simulink model "afe_dqctrl_inv_psm"  (R2026a)
settings: Solver=ode23t  StopTime=simlength  FixedStep=tc  MaxStep=glb_time.tc  RelTol=1e-4
values from neighbouring files (symbols this model uses):
  afe_ctrl = ctrl_afe_setup(glb_time.ts_afe, grid_emu.omega_grid_nom)    [init_model.m]
  afe_pwm_phase_shift_mod1 = 0    [init_model.m]
  CTRPIFF_CLIP_RELEASE = 0.001    [init_model.m]
  filters = setup_global_filters(glb_time.ts_afe, glb_time.ts_inv, glb_time.ts_dab, glb_time.tc)    [init_model.m]
  glb_time = timing_setup(fpwm_afe, trgo_afe, fpwm_inv, trgo_inv, fpwm_single_phase_inv, trgo_single_phase_inv, fpwm_dab, trgo_dab,      fpwm_psfbc, trgo_psfbc, fpwm_isop_rail, trgo_isop_rail, fpwm_cllc, trgo_cllc, t_measure, tc_factor, tc_decimation, delay_pwm, dead_time_afe,      dead_time_inv, dead_time_single_phase_inv, dead_time_dab, dead_time_psfbc, dead_time_isop_rail, dead_time_cllc)    [init_model.m]
  grid_emu = grid_three_phase_emulator('Dyn11', delta_star, grid_nominal_power, application_voltage, us1, us2, fgrid,                  eq_grid_inductance, eq_grid_resistance, eta, ucc, i1m, p_iron, n1, n2, core_area, core_length, mur,                  up_xi_pu_ref, up_eta_pu_ref, un_xi_pu_ref, un_eta_pu_ref)    [init_model.m]
  heatsink = liquid_cooled_plate_2kw_setup(weight, no_weight, cp_al, heat_capacity_hs, thermal_conductivity_al,      Rth_switch_HA, Rth_mosfet_HA, Rth_diode_HA, Tambient, DThs_init)    [init_model.m]
  inv_pwm_phase_shift_mod1 = 0    [init_model.m]
  ki_align = 18    [init_model.m]
  kp_align = 0.25    [init_model.m]
  lim_down_align = -0.05    [init_model.m]
  lim_up_align = 0.05    [init_model.m]
  omega_m_sim = psm.omega_m_bez    [init_model.m]
  psm = psm_calculus()    [init_model.m]
  psm_ctrl = ctrl_pmsm_setup(glb_time.ts_inv, psm.omega_bez, u_psm_scale, psm.Jm_norm)    [init_model.m]
  simlength = 1.75    [init_model.m]
  Tambient = 40    [init_model.m]
  time_gain_afe_module_1 = 1.0002    [init_model.m]
  time_gain_inv_module_2 = 1.001    [init_model.m]
  time_start_motor_control = 0.25    [init_model.m]
  torque_overload_factor = 1.15    [init_model.m]
  u_cm_comp_mod1 = 0    [init_model.m]
  u_psm_scale_ekf = sqrt(3)/2 * 2/3 * hwdata.inv.udc_nom/psm.ubez    [init_model.m]
undefined symbols (not defined in the file or in its folder): hwdata, igbt, magnitude, omega_m_bez, rpm_base, torque_base
libraries: fl_lib x99, nesl_utility x96, igbt_simple_lib x12, single_phase_transformer_lib x3, threephase_inductor_lib x2, dclink_for_two_levels x2, three_phase_pwm_modulator x2, cstblocks_lti x2, discrete_time_low_pass_filter x1, lithium_ion_battery x1, three_phase_voltage_with_frt_emulator x1, simple_flexible_shaft x1
(part 6 of 9)

== system afe_dqctrl_inv_psm/afe_dq_mod1/AFE_control/afe_control/grid_voltage_phase_lock_loops/dq_pll_ccaller/first_harmonic_tracker_phase_u ==
  u : Inport
  Bus Selector : BusSelector  OutputSignals=output_pu_hat
  C Caller : CCaller  FunctionName=first_harmonic_tracker_process_simulink  PortSpecificationStruct="%)30     .    B \\   8    (     @         %    \"     D    !     0         %  0 \"0    $    _    07)G3F%M90  4&]R=$YA;64 4V-O<&4     26YD97@     5'EP90      4VEZ90      27-';&]B86P   X    P    !@    @    $          4    (     0    ,    !         !   P!O=70 #@   #     &    \"     0         !0    @    !     P    $         $  # &]U=  .    .     8    (    !          %    \"     $    &     0         0  ...(+4988 chars)"
  Constant : Constant  Value=glb_time.ts_afe
  Constant1 : Constant  Value=0
  Constant4 : Constant  Value=afe_ctrl.fht_grid.omega_fht
  Constant5 : Constant  Value=afe_ctrl.fht_grid.delta_fht
  Constant6 : Constant  Value=afe_ctrl.fht_grid.Ld_fht(1)
  Constant7 : Constant  Value=afe_ctrl.fht_grid.Ld_fht(2)
  Data Type Conversion{1..2,6..9} (6 alike) : DataTypeConversion  OutDataTypeStr=single  SaturateOnIntegerOverflow=off  RndMeth=Floor
  Data Type Conversion3 : DataTypeConversion  OutDataTypeStr=uint8  SaturateOnIntegerOverflow=off  RndMeth=Floor
  Data Type Conversion4 : DataTypeConversion  OutDataTypeStr=double  SaturateOnIntegerOverflow=off  RndMeth=Floor
  Data Type Conversion5 : DataTypeConversion  OutDataTypeStr=uint8  SaturateOnIntegerOverflow=off  RndMeth=Floor
  Step : Step  Time=0.0125  InitialValue=1  FinalValue=0
  u_hat : Outport
  wires:
  Data Type Conversion4/1 -> u_hat/1
  Data Type Conversion3/1 -> C Caller/1
  Data Type Conversion1/1 -> C Caller/3
  Data Type Conversion2/1 -> C Caller/2
  C Caller/1 -> Bus Selector/1
  Bus Selector/1 -> Data Type Conversion4/1  "<output_pu_hat>"
  Step/1 -> Data Type Conversion3/1
  u/1 -> Data Type Conversion2/1
  Constant/1 -> Data Type Conversion1/1
  Constant1/1 -> Data Type Conversion5/1
  Constant4/1 -> Data Type Conversion6/1
  Constant6/1 -> Data Type Conversion8/1
  Constant7/1 -> Data Type Conversion9/1
  Constant5/1 -> Data Type Conversion7/1
  Data Type Conversion5/1 -> C Caller/8
  Data Type Conversion6/1 -> C Caller/4
  Data Type Conversion7/1 -> C Caller/5
  Data Type Conversion8/1 -> C Caller/6
  Data Type Conversion9/1 -> C Caller/7

== system afe_dqctrl_inv_psm/afe_dq_mod1/AFE_control/afe_control/grid_voltage_phase_lock_loops/dq_pll_ccaller/first_harmonic_tracker_phase_v ==
  u : Inport
  Bus Selector : BusSelector  OutputSignals=output_pu_hat
  C Caller : CCaller  FunctionName=first_harmonic_tracker_process_simulink  PortSpecificationStruct="%)30     .    B \\   8    (     @         %    \"     D    !     0         %  0 \"0    $    _    07)G3F%M90  4&]R=$YA;64 4V-O<&4     26YD97@     5'EP90      4VEZ90      27-';&]B86P   X    P    !@    @    $          4    (     0    ,    !         !   P!O=70 #@   #     &    \"     0         !0    @    !     P    $         $  # &]U=  .    .     8    (    !          %    \"     $    &     0         0  ...(+4988 chars)"
  Constant : Constant  Value=glb_time.ts_afe
  Constant1 : Constant  Value=2
  Constant4 : Constant  Value=afe_ctrl.fht_grid.omega_fht
  Constant5 : Constant  Value=afe_ctrl.fht_grid.delta_fht
  Constant6 : Constant  Value=afe_ctrl.fht_grid.Ld_fht(1)
  Constant7 : Constant  Value=afe_ctrl.fht_grid.Ld_fht(2)
  Data Type Conversion{1..2,6..9} (6 alike) : DataTypeConversion  OutDataTypeStr=single  SaturateOnIntegerOverflow=off  RndMeth=Floor
  Data Type Conversion3 : DataTypeConversion  OutDataTypeStr=uint8  SaturateOnIntegerOverflow=off  RndMeth=Floor
  Data Type Conversion4 : DataTypeConversion  OutDataTypeStr=double  SaturateOnIntegerOverflow=off  RndMeth=Floor
  Data Type Conversion5 : DataTypeConversion  OutDataTypeStr=uint8  SaturateOnIntegerOverflow=off  RndMeth=Floor
  Step : Step  Time=0.0125  InitialValue=1  FinalValue=0
  u_hat : Outport
  wires:
  Data Type Conversion9/1 -> C Caller/7
  Data Type Conversion8/1 -> C Caller/6
  Data Type Conversion7/1 -> C Caller/5
  Data Type Conversion6/1 -> C Caller/4
  Data Type Conversion5/1 -> C Caller/8
  Constant5/1 -> Data Type Conversion7/1
  Constant7/1 -> Data Type Conversion9/1
  Constant6/1 -> Data Type Conversion8/1
  Constant4/1 -> Data Type Conversion6/1
  Constant1/1 -> Data Type Conversion5/1
  Constant/1 -> Data Type Conversion1/1
  u/1 -> Data Type Conversion2/1
  Step/1 -> Data Type Conversion3/1
  Bus Selector/1 -> Data Type Conversion4/1  "<output_pu_hat>"
  C Caller/1 -> Bus Selector/1
  Data Type Conversion2/1 -> C Caller/2
  Data Type Conversion1/1 -> C Caller/3
  Data Type Conversion3/1 -> C Caller/1
  Data Type Conversion4/1 -> u_hat/1

== system afe_dqctrl_inv_psm/afe_dq_mod1/AFE_control/afe_control/grid_voltage_phase_lock_loops/dq_pll_ccaller/first_harmonic_tracker_phase_w ==
  u : Inport
  Bus Selector : BusSelector  OutputSignals=output_pu_hat
  C Caller : CCaller  FunctionName=first_harmonic_tracker_process_simulink  PortSpecificationStruct="%)30     .    B \\   8    (     @         %    \"     D    !     0         %  0 \"0    $    _    07)G3F%M90  4&]R=$YA;64 4V-O<&4     26YD97@     5'EP90      4VEZ90      27-';&]B86P   X    P    !@    @    $          4    (     0    ,    !         !   P!O=70 #@   #     &    \"     0         !0    @    !     P    $         $  # &]U=  .    .     8    (    !          %    \"     $    &     0         0  ...(+4988 chars)"
  Constant : Constant  Value=glb_time.ts_afe
  Constant1 : Constant  Value=4
  Constant4 : Constant  Value=afe_ctrl.fht_grid.omega_fht
  Constant5 : Constant  Value=afe_ctrl.fht_grid.delta_fht
  Constant6 : Constant  Value=afe_ctrl.fht_grid.Ld_fht(1)
  Constant7 : Constant  Value=afe_ctrl.fht_grid.Ld_fht(2)
  Data Type Conversion{1..2,6..9} (6 alike) : DataTypeConversion  OutDataTypeStr=single  SaturateOnIntegerOverflow=off  RndMeth=Floor
  Data Type Conversion3 : DataTypeConversion  OutDataTypeStr=uint8  SaturateOnIntegerOverflow=off  RndMeth=Floor
  Data Type Conversion4 : DataTypeConversion  OutDataTypeStr=double  SaturateOnIntegerOverflow=off  RndMeth=Floor
  Data Type Conversion5 : DataTypeConversion  OutDataTypeStr=uint8  SaturateOnIntegerOverflow=off  RndMeth=Floor
  Step : Step  Time=0.0125  InitialValue=1  FinalValue=0
  u_hat : Outport
  wires:
  Data Type Conversion4/1 -> u_hat/1
  Data Type Conversion3/1 -> C Caller/1
  Data Type Conversion1/1 -> C Caller/3
  Data Type Conversion2/1 -> C Caller/2
  C Caller/1 -> Bus Selector/1
  Bus Selector/1 -> Data Type Conversion4/1  "<output_pu_hat>"
  Step/1 -> Data Type Conversion3/1
  u/1 -> Data Type Conversion2/1
  Constant/1 -> Data Type Conversion1/1
  Constant1/1 -> Data Type Conversion5/1
  Constant4/1 -> Data Type Conversion6/1
  Constant6/1 -> Data Type Conversion8/1
  Constant7/1 -> Data Type Conversion9/1
  Constant5/1 -> Data Type Conversion7/1
  Data Type Conversion5/1 -> C Caller/8
  Data Type Conversion6/1 -> C Caller/4
  Data Type Conversion7/1 -> C Caller/5
  Data Type Conversion8/1 -> C Caller/6
  Data Type Conversion9/1 -> C Caller/7

== system afe_dqctrl_inv_psm/afe_dq_mod1/afe/three_phase_inverter_with_igbt_simple/three_phase_inverter_with_igbt_simple/igbt_simple_1/IGBT_simple ==
  IGBT_SIMPLE Simplified IGBT + antiparallel FWD : igbt_simple_lib/IGBT_SIMPLE Simplified IGBT + antiparallel FWD  Vce_sat=vce_sat_m V  Vf=v_gamma_m V  Vth=Vth_gate_m V  Vhyst=Vth_gate_hyst_m V  Ron=rce_on_m mOhm  Rd=rd_on_m mOhm  Goff=Gce_off_m 1/Ohm  i_specify=off  i_priority=None  i=0 A  i_nominal_specify=off  i_nominal_value=1  i_nominal_unit=A  v_specify=off  v_priority=None  v=0 V  v_nominal_specify=off  v_nominal_value=1  v_nominal_unit=V  i_t_specify=off  i_t_priority=None  i_t=0 A  i_t_nominal_specify=off  i_t_nominal_value=1  i_t_nominal_unit=A  i_d_specify=off  i_d_priority=None  i_d=0 A  i_d_nominal_specify=off  i_d_nominal_value=1  i_d_nominal_unit=A
  iph1 : nesl_utility/PS-Simulink Converter  PhysicalDomain=network_engine_domain  SubClassName=ps_output  LeftPortType=input  RightPortType=output  PseudoPeriodic=off  Frequencies=[]  VectorFormat=1-D array  Unit=A  AffineConversion=off
  iph2 : nesl_utility/PS-Simulink Converter  PhysicalDomain=network_engine_domain  SubClassName=ps_output  LeftPortType=input  RightPortType=output  PseudoPeriodic=off  Frequencies=[]  VectorFormat=1-D array  Unit=A  AffineConversion=off
  G : PMIOPort  Side=Left
  C : PMIOPort  Port=2  Side=Left
  E : PMIOPort  Port=3  Side=Right
  tag scope: diode_current_Q1=scoped, igbt_current_Q1=scoped
  wires:
  iph1/1 -> [igbt_current_Q1]  "i_device_thermal_inv"
  iph2/1 -> [diode_current_Q1]  "i_device_thermal_inv"
  connections:
  IGBT_SIMPLE Simplified IGBT + antiparallel FWD/RConn1 -- E/RConn1
  IGBT_SIMPLE Simplified IGBT + antiparallel FWD/LConn1 -- C/RConn1
  IGBT_SIMPLE Simplified IGBT + antiparallel FWD/LConn2 -- G/RConn1
  IGBT_SIMPLE Simplified IGBT + antiparallel FWD/RConn2 -- iph1/LConn1
  IGBT_SIMPLE Simplified IGBT + antiparallel FWD/RConn3 -- iph2/LConn1

== system afe_dqctrl_inv_psm/afe_dq_mod1/afe/three_phase_inverter_with_igbt_simple/three_phase_inverter_with_igbt_simple/igbt_simple_2/IGBT_simple ==
  IGBT_SIMPLE Simplified IGBT + antiparallel FWD : igbt_simple_lib/IGBT_SIMPLE Simplified IGBT + antiparallel FWD  Vce_sat=vce_sat_m V  Vf=v_gamma_m V  Vth=Vth_gate_m V  Vhyst=Vth_gate_hyst_m V  Ron=rce_on_m mOhm  Rd=rd_on_m mOhm  Goff=Gce_off_m 1/Ohm  i_specify=off  i_priority=None  i=0 A  i_nominal_specify=off  i_nominal_value=1  i_nominal_unit=A  v_specify=off  v_priority=None  v=0 V  v_nominal_specify=off  v_nominal_value=1  v_nominal_unit=V  i_t_specify=off  i_t_priority=None  i_t=0 A  i_t_nominal_specify=off  i_t_nominal_value=1  i_t_nominal_unit=A  i_d_specify=off  i_d_priority=None  i_d=0 A  i_d_nominal_specify=off  i_d_nominal_value=1  i_d_nominal_unit=A
  iph1 : nesl_utility/PS-Simulink Converter  PhysicalDomain=network_engine_domain  SubClassName=ps_output  LeftPortType=input  RightPortType=output  PseudoPeriodic=off  Frequencies=[]  VectorFormat=1-D array  Unit=A  AffineConversion=off
  iph2 : nesl_utility/PS-Simulink Converter  PhysicalDomain=network_engine_domain  SubClassName=ps_output  LeftPortType=input  RightPortType=output  PseudoPeriodic=off  Frequencies=[]  VectorFormat=1-D array  Unit=A  AffineConversion=off
  G : PMIOPort  Side=Left
  C : PMIOPort  Port=2  Side=Left
  E : PMIOPort  Port=3  Side=Right
  tag scope: diode_current_Q2=scoped, igbt_current_Q2=scoped
  wires:
  iph1/1 -> [igbt_current_Q2]  "i_device_thermal_inv"
  iph2/1 -> [diode_current_Q2]  "i_device_thermal_inv"
  connections:
  IGBT_SIMPLE Simplified IGBT + antiparallel FWD/RConn1 -- E/RConn1
  IGBT_SIMPLE Simplified IGBT + antiparallel FWD/LConn1 -- C/RConn1
  IGBT_SIMPLE Simplified IGBT + antiparallel FWD/LConn2 -- G/RConn1
  IGBT_SIMPLE Simplified IGBT + antiparallel FWD/RConn2 -- iph1/LConn1
  IGBT_SIMPLE Simplified IGBT + antiparallel FWD/RConn3 -- iph2/LConn1

== system afe_dqctrl_inv_psm/afe_dq_mod1/afe/three_phase_inverter_with_igbt_simple/three_phase_inverter_with_igbt_simple/igbt_simple_3/IGBT_simple ==
  IGBT_SIMPLE Simplified IGBT + antiparallel FWD : igbt_simple_lib/IGBT_SIMPLE Simplified IGBT + antiparallel FWD  Vce_sat=vce_sat_m V  Vf=v_gamma_m V  Vth=Vth_gate_m V  Vhyst=Vth_gate_hyst_m V  Ron=rce_on_m mOhm  Rd=rd_on_m mOhm  Goff=Gce_off_m 1/Ohm  i_specify=off  i_priority=None  i=0 A  i_nominal_specify=off  i_nominal_value=1  i_nominal_unit=A  v_specify=off  v_priority=None  v=0 V  v_nominal_specify=off  v_nominal_value=1  v_nominal_unit=V  i_t_specify=off  i_t_priority=None  i_t=0 A  i_t_nominal_specify=off  i_t_nominal_value=1  i_t_nominal_unit=A  i_d_specify=off  i_d_priority=None  i_d=0 A  i_d_nominal_specify=off  i_d_nominal_value=1  i_d_nominal_unit=A
  iph1 : nesl_utility/PS-Simulink Converter  PhysicalDomain=network_engine_domain  SubClassName=ps_output  LeftPortType=input  RightPortType=output  PseudoPeriodic=off  Frequencies=[]  VectorFormat=1-D array  Unit=A  AffineConversion=off
  iph2 : nesl_utility/PS-Simulink Converter  PhysicalDomain=network_engine_domain  SubClassName=ps_output  LeftPortType=input  RightPortType=output  PseudoPeriodic=off  Frequencies=[]  VectorFormat=1-D array  Unit=A  AffineConversion=off
  G : PMIOPort  Side=Left
  C : PMIOPort  Port=2  Side=Left
  E : PMIOPort  Port=3  Side=Right
  tag scope: diode_current_Q3=scoped, igbt_current_Q3=scoped
  wires:
  iph1/1 -> [igbt_current_Q3]  "i_device_thermal_inv"
  iph2/1 -> [diode_current_Q3]  "i_device_thermal_inv"
  connections:
  IGBT_SIMPLE Simplified IGBT + antiparallel FWD/RConn1 -- E/RConn1
  IGBT_SIMPLE Simplified IGBT + antiparallel FWD/LConn1 -- C/RConn1
  IGBT_SIMPLE Simplified IGBT + antiparallel FWD/LConn2 -- G/RConn1
  IGBT_SIMPLE Simplified IGBT + antiparallel FWD/RConn2 -- iph1/LConn1
  IGBT_SIMPLE Simplified IGBT + antiparallel FWD/RConn3 -- iph2/LConn1

== system afe_dqctrl_inv_psm/afe_dq_mod1/afe/three_phase_inverter_with_igbt_simple/three_phase_inverter_with_igbt_simple/igbt_simple_4/IGBT_simple ==
  IGBT_SIMPLE Simplified IGBT + antiparallel FWD : igbt_simple_lib/IGBT_SIMPLE Simplified IGBT + antiparallel FWD  Vce_sat=vce_sat_m V  Vf=v_gamma_m V  Vth=Vth_gate_m V  Vhyst=Vth_gate_hyst_m V  Ron=rce_on_m mOhm  Rd=rd_on_m mOhm  Goff=Gce_off_m 1/Ohm  i_specify=off  i_priority=None  i=0 A  i_nominal_specify=off  i_nominal_value=1  i_nominal_unit=A  v_specify=off  v_priority=None  v=0 V  v_nominal_specify=off  v_nominal_value=1  v_nominal_unit=V  i_t_specify=off  i_t_priority=None  i_t=0 A  i_t_nominal_specify=off  i_t_nominal_value=1  i_t_nominal_unit=A  i_d_specify=off  i_d_priority=None  i_d=0 A  i_d_nominal_specify=off  i_d_nominal_value=1  i_d_nominal_unit=A
  iph1 : nesl_utility/PS-Simulink Converter  PhysicalDomain=network_engine_domain  SubClassName=ps_output  LeftPortType=input  RightPortType=output  PseudoPeriodic=off  Frequencies=[]  VectorFormat=1-D array  Unit=A  AffineConversion=off
  iph2 : nesl_utility/PS-Simulink Converter  PhysicalDomain=network_engine_domain  SubClassName=ps_output  LeftPortType=input  RightPortType=output  PseudoPeriodic=off  Frequencies=[]  VectorFormat=1-D array  Unit=A  AffineConversion=off
  G : PMIOPort  Side=Left
  C : PMIOPort  Port=2  Side=Left
  E : PMIOPort  Port=3  Side=Right
  tag scope: diode_current_Q4=scoped, igbt_current_Q4=scoped
  wires:
  iph1/1 -> [igbt_current_Q4]  "i_device_thermal_inv"
  iph2/1 -> [diode_current_Q4]  "i_device_thermal_inv"
  connections:
  IGBT_SIMPLE Simplified IGBT + antiparallel FWD/RConn1 -- E/RConn1
  IGBT_SIMPLE Simplified IGBT + antiparallel FWD/LConn1 -- C/RConn1
  IGBT_SIMPLE Simplified IGBT + antiparallel FWD/LConn2 -- G/RConn1
  IGBT_SIMPLE Simplified IGBT + antiparallel FWD/RConn2 -- iph1/LConn1
  IGBT_SIMPLE Simplified IGBT + antiparallel FWD/RConn3 -- iph2/LConn1

== system afe_dqctrl_inv_psm/afe_dq_mod1/afe/three_phase_inverter_with_igbt_simple/three_phase_inverter_with_igbt_simple/igbt_simple_5/IGBT_simple ==
  IGBT_SIMPLE Simplified IGBT + antiparallel FWD : igbt_simple_lib/IGBT_SIMPLE Simplified IGBT + antiparallel FWD  Vce_sat=vce_sat_m V  Vf=v_gamma_m V  Vth=Vth_gate_m V  Vhyst=Vth_gate_hyst_m V  Ron=rce_on_m mOhm  Rd=rd_on_m mOhm  Goff=Gce_off_m 1/Ohm  i_specify=off  i_priority=None  i=0 A  i_nominal_specify=off  i_nominal_value=1  i_nominal_unit=A  v_specify=off  v_priority=None  v=0 V  v_nominal_specify=off  v_nominal_value=1  v_nominal_unit=V  i_t_specify=off  i_t_priority=None  i_t=0 A  i_t_nominal_specify=off  i_t_nominal_value=1  i_t_nominal_unit=A  i_d_specify=off  i_d_priority=None  i_d=0 A  i_d_nominal_specify=off  i_d_nominal_value=1  i_d_nominal_unit=A
  iph1 : nesl_utility/PS-Simulink Converter  PhysicalDomain=network_engine_domain  SubClassName=ps_output  LeftPortType=input  RightPortType=output  PseudoPeriodic=off  Frequencies=[]  VectorFormat=1-D array  Unit=A  AffineConversion=off
  iph2 : nesl_utility/PS-Simulink Converter  PhysicalDomain=network_engine_domain  SubClassName=ps_output  LeftPortType=input  RightPortType=output  PseudoPeriodic=off  Frequencies=[]  VectorFormat=1-D array  Unit=A  AffineConversion=off
  G : PMIOPort  Side=Left
  C : PMIOPort  Port=2  Side=Left
  E : PMIOPort  Port=3  Side=Right
  tag scope: diode_current_Q5=scoped, igbt_current_Q5=scoped
  wires:
  iph1/1 -> [igbt_current_Q5]  "i_device_thermal_inv"
  iph2/1 -> [diode_current_Q5]  "i_device_thermal_inv"
  connections:
  IGBT_SIMPLE Simplified IGBT + antiparallel FWD/RConn1 -- E/RConn1
  IGBT_SIMPLE Simplified IGBT + antiparallel FWD/LConn1 -- C/RConn1
  IGBT_SIMPLE Simplified IGBT + antiparallel FWD/LConn2 -- G/RConn1
  IGBT_SIMPLE Simplified IGBT + antiparallel FWD/RConn2 -- iph1/LConn1
  IGBT_SIMPLE Simplified IGBT + antiparallel FWD/RConn3 -- iph2/LConn1

== system afe_dqctrl_inv_psm/afe_dq_mod1/afe/three_phase_inverter_with_igbt_simple/three_phase_inverter_with_igbt_simple/igbt_simple_6/IGBT_simple ==
  IGBT_SIMPLE Simplified IGBT + antiparallel FWD : igbt_simple_lib/IGBT_SIMPLE Simplified IGBT + antiparallel FWD  Vce_sat=vce_sat_m V  Vf=v_gamma_m V  Vth=Vth_gate_m V  Vhyst=Vth_gate_hyst_m V  Ron=rce_on_m mOhm  Rd=rd_on_m mOhm  Goff=Gce_off_m 1/Ohm  i_specify=off  i_priority=None  i=0 A  i_nominal_specify=off  i_nominal_value=1  i_nominal_unit=A  v_specify=off  v_priority=None  v=0 V  v_nominal_specify=off  v_nominal_value=1  v_nominal_unit=V  i_t_specify=off  i_t_priority=None  i_t=0 A  i_t_nominal_specify=off  i_t_nominal_value=1  i_t_nominal_unit=A  i_d_specify=off  i_d_priority=None  i_d=0 A  i_d_nominal_specify=off  i_d_nominal_value=1  i_d_nominal_unit=A
  iph1 : nesl_utility/PS-Simulink Converter  PhysicalDomain=network_engine_domain  SubClassName=ps_output  LeftPortType=input  RightPortType=output  PseudoPeriodic=off  Frequencies=[]  VectorFormat=1-D array  Unit=A  AffineConversion=off
  iph2 : nesl_utility/PS-Simulink Converter  PhysicalDomain=network_engine_domain  SubClassName=ps_output  LeftPortType=input  RightPortType=output  PseudoPeriodic=off  Frequencies=[]  VectorFormat=1-D array  Unit=A  AffineConversion=off
  G : PMIOPort  Side=Left
  C : PMIOPort  Port=2  Side=Left
  E : PMIOPort  Port=3  Side=Right
  tag scope: diode_current_Q6=scoped, igbt_current_Q6=scoped
  wires:
  iph1/1 -> [igbt_current_Q6]  "i_device_thermal_inv"
  iph2/1 -> [diode_current_Q6]  "i_device_thermal_inv"
  connections:
  IGBT_SIMPLE Simplified IGBT + antiparallel FWD/RConn1 -- E/RConn1
  IGBT_SIMPLE Simplified IGBT + antiparallel FWD/LConn1 -- C/RConn1
  IGBT_SIMPLE Simplified IGBT + antiparallel FWD/LConn2 -- G/RConn1
  IGBT_SIMPLE Simplified IGBT + antiparallel FWD/RConn2 -- iph1/LConn1
  IGBT_SIMPLE Simplified IGBT + antiparallel FWD/RConn3 -- iph2/LConn1

== system afe_dqctrl_inv_psm/inv_dq_mod1/INV_control/inverter_control/current_ctrl/bemf_observer/EKF_bemf_observer ==
  ialpha_pu : Inport
  ibeta_pu : Inport  Port=2
  ualpha_pu : Inport  Port=3
  ubeta_pu : Inport  Port=4
  udc_pu : Inport  Port=5
  EKF Observer simulink/Ccaller mod1 : Scope  NumInputPorts=2
      settings: ActiveDisplayYMinimum=-3.9268483156565956  ActiveDisplayYMaximum=3.9269848822951774
  Gain : Gain  Gain=u_psm_scale_ekf
  Gain1 : Gain  Gain=u_psm_scale_ekf
  Mux{,1..3} (4 alike) : Mux  Inputs=2
  Terminator : Terminator
  extended_kalman_observer : Subsystem
  phase_elec_ekf_hat : Outport
  omega_elec_ekf_hat : Outport  Port=2
  tag scope: psi_r_alpha_hat_mod1=scoped, psi_r_beta_hat_mod1=scoped
  wires:
  ialpha_pu/1 -> Mux2/1
  ibeta_pu/1 -> Mux2/2
  Mux/1 -> EKF Observer simulink/Ccaller mod1/1
  Mux1/1 -> EKF Observer simulink/Ccaller mod1/2
  extended_kalman_observer/3(phase_elec_ekf_hat) -> phase_elec_ekf_hat/1, Mux1/1  "phase_elec_ekf_hat"
  extended_kalman_observer/4(omega_elec_ekf_hat) -> omega_elec_ekf_hat/1, Mux/1  "omega_elec_ekf_hat"
  [omegad_pu_psm] -> Mux/2  "omega_pu_psm_encoder"
  [phased_psm] -> Mux1/2  "phase_psm_encoder"
  udc_pu/1 -> Terminator/1
  extended_kalman_observer/1(psi_alpha_ekf_hat) -> [psi_r_alpha_hat_mod1]
  extended_kalman_observer/2(psi_beta_ekf_hat) -> [psi_r_beta_hat_mod1]
  Mux2/1 -> extended_kalman_observer/2(ialphabeta)
  Mux3/1 -> extended_kalman_observer/1(ualphabeta)
  Gain/1 -> Mux3/1
  Gain1/1 -> Mux3/2
  ualpha_pu/1 -> Gain/1
  ubeta_pu/1 -> Gain1/1

== system afe_dqctrl_inv_psm/inv_dq_mod1/INV_control/inverter_control/current_ctrl/bemf_observer/bemf_observer ==
  ialpha_pu : Inport
  ibeta_pu : Inport  Port=2
  ualpha_pu : Inport  Port=3
  ubeta_pu : Inport  Port=4
  udc_pu : Inport  Port=5
  Gain : Gain  Gain=psm.psi_m_norm
  Gain1 : Gain  Gain=psm.psi_m_norm
  Goto Tag Visibility : GotoTagVisibility  GotoTag=psi_r_alpha_hat_mod1
  Goto Tag Visibility1 : GotoTagVisibility  GotoTag=psi_r_beta_hat_mod1
  Goto Tag Visibility2 : GotoTagVisibility  GotoTag=theta_bemf_hat_mod1
  Goto Tag Visibility3 : GotoTagVisibility  GotoTag=psi_r_m_alpha_mod1
  Goto Tag Visibility4 : GotoTagVisibility  GotoTag=psi_r_m_beta_mod1
  Trigonometric Function : Trigonometry  Operator=cos
  Trigonometric Function1 : Trigonometry
  double_integrator_observer : Subsystem
  psi_alpha_hat : Subsystem
  psi_beta_hat : Subsystem
  theta_bemf_hat : Subsystem
  omega_pu : Outport
  theta_hat : Outport  Port=2
  tag scope: psi_r_alpha_hat_mod1=scoped, psi_r_alpha_pu_hat_mod1=scoped, psi_r_beta_hat_mod1=scoped, psi_r_beta_pu_hat_mod1=scoped, psi_r_m_alpha_mod1=scoped, psi_r_m_beta_mod1=scoped, theta_bemf_hat_mod1=scoped
  wires:
  Trigonometric Function/1 -> Gain/1
  Trigonometric Function1/1 -> Gain1/1
  ialpha_pu/1 -> psi_alpha_hat/2(ialpha)
  ibeta_pu/1 -> psi_beta_hat/2(ibeta)
  psi_alpha_hat/2(psi_r_alpha_hat) -> [psi_r_alpha_hat_mod1]
  psi_beta_hat/2(psi_r_beta_hat) -> [psi_r_beta_hat_mod1]
  [psi_r_alpha_hat_mod1] -> theta_bemf_hat/1(psi_r_alpha_hat)
  [psi_r_beta_hat_mod1] -> theta_bemf_hat/2(psi_r_beta_hat)
  ualpha_pu/1 -> psi_alpha_hat/1(ualpha)
  ubeta_pu/1 -> psi_beta_hat/1(ubeta)
  [phase_hat_mod1] -> Trigonometric Function/1, Trigonometric Function1/1
  Gain/1 -> [psi_r_m_alpha_mod1]
  Gain1/1 -> [psi_r_m_beta_mod1]
  theta_bemf_hat/1(theta_emf_hat) -> [theta_bemf_hat_mod1]
  [theta_bemf_hat_mod1] -> double_integrator_observer/1(theta)
  double_integrator_observer/1(omega_pu_hat) -> omega_pu/1
  double_integrator_observer/2(theta_hat) -> theta_hat/1
  [psi_r_alpha_hat_mod1] -> [psi_r_alpha_pu_hat_mod1]
  [psi_r_beta_hat_mod1] -> [psi_r_beta_pu_hat_mod1]
  udc_pu/1 -> psi_alpha_hat/3(udc), psi_beta_hat/3(udc)
